simulink model "InfusionPumpSoftwareModelNoOccDetect"  (R2022b)
settings: Solver=FixedStepDiscrete  StartTime=0.0  StopTime=120  FixedStep=0.001  MaxStep=0.001  RelTol=1e-5
undefined symbols (not defined in the file): reserv_str
settings Model: Creator=szhang  LastModifiedBy=ppatel
settings SolverCC: AlgebraicLoopSolver=TrustRegion
settings DataIOCC: InitialState=simState  LimitDataPoints=on  SaveFinalState=on  SaveOutput=off  SaveTime=off
settings OptimizationCC: DefaultParameterBehavior=Inlined  UseDivisionForNetSlopeComputation=on  UseFloatMulNetSlope=on  InlineInvariantSignals=on  PassReuseOutputArgsAs=Individual arguments  ZeroExternalMemoryAtStartup=off  ZeroInternalMemoryAtStartup=off  NoFixptDivByZeroProtection=on  EfficientFloat2IntCast=on  LifeSpan=1  EfficientTunableParamExpr=on
settings DebuggingCC: SignalRangeChecking=error  SolverPrmCheckMsg=warning  IntegerOverflowMsg=error  ParameterTunabilityLossMsg=error  UnconnectedInputMsg=warning  UnconnectedOutputMsg=warning  UnconnectedLineMsg=warning  SFUnexpectedBacktrackingDiag=warning  SFNoUnconditionalDefaultTransitionDiag=warning  SFUnreachableExecutionPathDiag=error  SFExecutionAtInitializationDiag=none  SFMachineParentedDataDiag=warning  ArithmeticOperatorsInVariantConditions=warning
settings HardwareCC: ProdLongLongMode=on
settings ModelReferenceCC: EnableRefExpFcnMdlSchedulingChecks=on  PropagateVarSize=During execution  PropagateSignalLabelsOutOfModel=off
settings SFSimCC: SimUseLocalCustomCode=off  CustomCodeUndefinedFunction=UseInterfaceOnly
settings RTWCC: Description=Embedded Coder  SystemTargetFile=ert.tlc  TemplateMakefile=ert_default_tmf  GenerateReport=on  RTWUseLocalCustomCode=off  IncludeHyperlinkInReport=on  LaunchReport=on  PortableWordSizes=on  GenerateTraceInfo=on  GenerateTraceReport=on  GenerateTraceReportSl=on  GenerateTraceReportSf=on  GenerateTraceReportEml=on  GenerateCodeMetricsReport=on
settings CodeAppCC: ForceParamTrailComments=on  IgnoreCustomStorageClasses=off  OperatorAnnotations=on  SimulinkDataObjDesc=on  SFDataObjDesc=on  MATLABFcnDesc=on  CustomSymbolStrGlobalVar=rt$N$M  CustomSymbolStrType=$N$M  CustomSymbolStrFcn=$N$M$F  CustomSymbolStrMacro=$N$M  InsertBlockDesc=on  StateflowObjectComments=on  MATLABSourceComments=on  ReqsInCode=on
settings ERTTargetCC: MultiwordLength=2048  GenerateSampleERTMain=on  CombineSignalStateStructs=on  SupportAbsoluteTime=off  SupportComplex=off  InlinedParameterPlacement=NonHierarchical  ERTCustomFileTemplate=example_file_process.tlc  ERTFilePackagingFormat=CompactWithDataFile
settings ConfigComp: CovEnable=on  RecordCoverage=on  CovMetricSettings=dcmw  CovHTMLOptions=-sRT=1 -sVT=0 -aTS=1 -bRG=1 -bTC=1 -hTR=0 -nFC=0 -nFD=1 -scm=1 -bcm=1 -xEv=0 -xEM=0  CovSaveCumulativeToWorkspaceVar=on  CovSaveSingleToWorkspaceVar=on  CovCumulativeReport=on  CovModelRefEnable=on  CovExternalEMLEnable=off  CovSFcnEnable=off  DVTestSuiteOptimization=CombinedObjectives (Nonlinear Extended)  DVDesignMinMaxCheck=on  DVHarnessSource=Signal Editor  PSOpenProjectManager=on  PSResultDir=ps_results_$ModelName$  PSAutoStubLUT=on
settings SimscapeCC: SimscapeNormalizeSystem=off  SimscapeNominalValues="[{\"value\":\"10\",\"unit\":\"V\"},{\"value\":\"1\",\"unit\":\"A\"},{\"value\":\"10\",\"unit\":\"N*m\"},{\"value\":\"10\",\"unit\":\"bar\"},{\"value\":\"100\",\"unit\":\"kJ/kg\"},{\"value\":\"1\",\"unit\":\"kW\"},{\"value\":\"300\",\"unit\":\"K\"},{\"value\":\"100\",\"unit\":\"cm^3/s\"},{\"value\":\"1\",\"unit\":\"kN\"},{\"value\":\"1\",\"unit\":\"g/cm^3\"},{\"value\":\"1\",\"unit\":\"l\"},{\"value\":\"1\",\"unit\":\"cm^2\"},{\"value\":\"60\",\"unit\":\"Hz\"}]"  SimscapeLogType=all  SimscapeLogLimitData=off

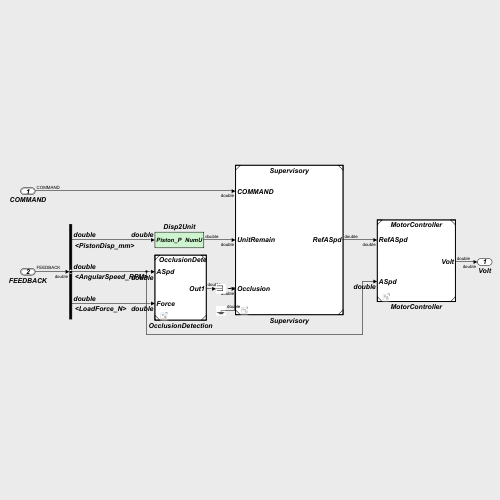
[thumbnail: Simulink's stored preview of the top-level diagram]
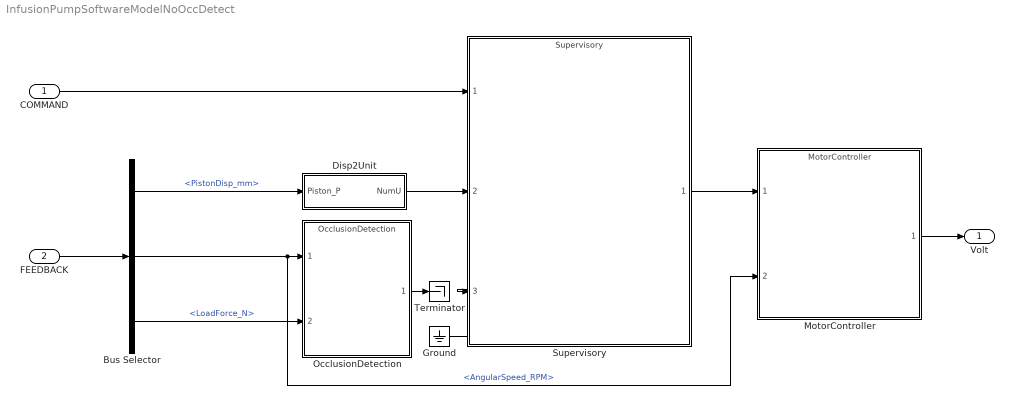
== system InfusionPumpSoftwareModelNoOccDetect ==
  COMMAND : Inport  OutDataTypeStr=Bus: COMMAND  SampleTime=0.001  BusOutputAsStruct=on
  FEEDBACK : Inport  Port=2  OutDataTypeStr=Bus: FEEDBACK  SampleTime=0.001  BusOutputAsStruct=on
  Bus Selector : BusSelector  OutputSignals=PistonDisp_mm,AngularSpeed_RPM,LoadForce_N
  Disp2Unit : Subsystem
  Ground : Ground
  MotorController : ModelReference  ModelNameDialog=MotorController  SimulationMode=Normal  ModelReferenceVersion=11.6
  OcclusionDetection : ModelReference  ModelNameDialog=OcclusionDetection.slx  SimulationMode=Normal  ModelReferenceVersion=9.8
  Supervisory : ModelReference  ModelNameDialog=Supervisory  SimulationMode=Normal  ModelReferenceVersion=11.11
  Terminator : Terminator
  Volt : Outport  OutMin=-10  OutMax=10  OutDataTypeStr=double  PortDimensions=1  SampleTime=[0.001,0]
  wires:
  Disp2Unit/1(NumU) -> Supervisory/2
  Supervisory/1 -> MotorController/1
  Bus Selector/2 -> MotorController/2, OcclusionDetection/1  "<AngularSpeed_RPM>"
  MotorController/1 -> Volt/1
  Bus Selector/3 -> OcclusionDetection/2  "<LoadForce_N>"
  FEEDBACK/1 -> Bus Selector/1
  Bus Selector/1 -> Disp2Unit/1(Piston_P)  "<PistonDisp_mm>"
  COMMAND/1 -> Supervisory/1
  OcclusionDetection/1 -> Terminator/1
  Ground/1 -> Supervisory/3

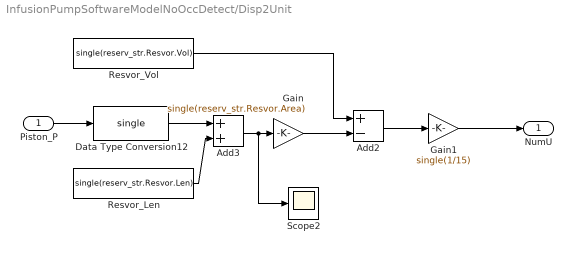
== system InfusionPumpSoftwareModelNoOccDetect/Disp2Unit ==
  Piston_P : Inport  OutMin=-30  OutMax=0
  Add2 : Sum  Inputs=+-
  Add3 : Sum
  Data Type Conversion12 : DataTypeConversion  OutDataTypeStr=single  SaturateOnIntegerOverflow=off  RndMeth=Floor
  Gain : Gain  Gain=single(reserv_str.Resvor.Area)
  Gain1 : Gain  Gain=single(1/15)
  Resvor_Len : Constant  Value=single(reserv_str.Resvor.Len)  OutDataTypeStr=single
  Resvor_Vol : Constant  Value=single(reserv_str.Resvor.Vol)  OutDataTypeStr=single
  Scope2 : Scope
  NumU : Outport  OutMin=0  OutMax=201
  wires:
  Resvor_Vol/1 -> Add2/1
  Resvor_Len/1 -> Add3/2
  Gain/1 -> Add2/2
  Add2/1 -> Gain1/1
  Gain1/1 -> NumU/1
  Add3/1 -> Gain/1, Scope2/1
  Piston_P/1 -> Data Type Conversion12/1
  Data Type Conversion12/1 -> Add3/1
